simulink model "VSDk_PMSM_6"  (R2024a)
settings: Solver=VariableStepAuto  StartTime=0.0  StopTime=10.0  RelTol=1e-3
values from neighbouring files (symbols this model uses):
  faif = 0.1351    [init.m]
  Iq_limit = Tn/(1.5*p*faif)*1    (= 90.6192943499)    [init.m]
  Jm = 0.36    [init.m]
  Ki_id_vsd = Rs * wc    (= 61.7197292724)    [init.m]
  Ki_iq_vsd = Rs * wc    (= 61.7197292724)    [init.m]
  Ki_x = Rs * wc_xy    (= 61.7197292724)    [init.m]
  Ki_y = Rs * wc_xy    (= 61.7197292724)    [init.m]
  Kis_vsd = (ws^2 * Jm) / KT    (= 438.324399752)    [init.m]
  Kp_id_vsd = Ld_eff * wc    (= 0.485061905714)    [init.m]
  Kp_iq_vsd = Lq_eff * wc    (= 0.485061905714)    [init.m]
  Kp_x = Lx * wc_xy    (= 0.020106192983)    [init.m]
  Kp_y = Ly * wc_xy    (= 0.020106192983)    [init.m]
  Kps_vsd = (2 * zeta * ws * Jm) / KT    (= 19.7285507573)    [init.m]
  LD = Ld+Ldd    (= 7.72e-05)    [init.m]
  Ld = 40.2e-6    (= 4.02e-05)    [init.m]
  Ldd = 37e-6    (= 3.7e-05)    [init.m]
  Ldz = Ld-Ldd    (= 3.2e-06)    [init.m]
  LQ = Lq+Lqq    (= 7.72e-05)    [init.m]
  Lq = 40.2e-6    (= 4.02e-05)    [init.m]
  Lqq = 37e-6    (= 3.7e-05)    [init.m]
  n = 2000    [init.m]
  p = 4    [init.m]
  Rs = 9.823e-3    (= 0.009823)    [init.m]
  Tn = 734.56/10    (= 73.456)    [init.m]
  Ts = 1/(16e3)    (= 6.25e-05)    [init.m]
  Ts_FEA = 1e-7    (= 1e-07)    [init.m]
  VDC = 1200    [init.m]
  wc_xy = 2 * pi * fc_xy    (= 6283.18530718)    [init.m]
libraries: spsIGBTDiodeLib x24, spsVoltageMeasurementLib x16, spsSeriesRLCBranchLib x12, spsDiodeLib x12, spsOnDelayLib x12, slpidlib x11, simulink x7, spsControlledCurrentSourceLib x6, spsDCVoltageSourceLib x1, spsdq0toAlphaBetaZeroLib x1, spspowerguiLib x1
(part 2 of 3)

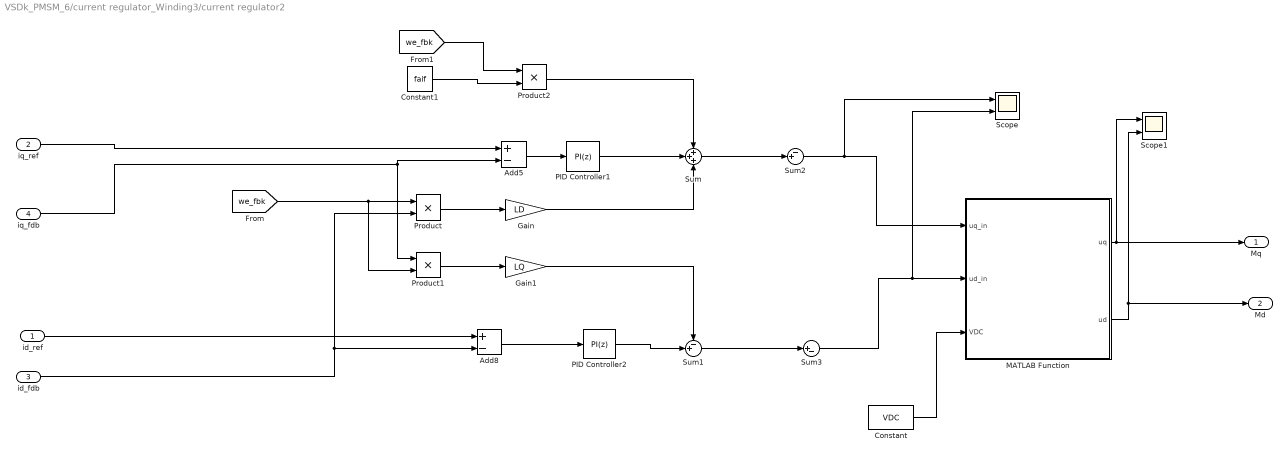
== system VSDk_PMSM_6/current regulator_Winding3/current regulator2 ==
  id_ref : Inport
  iq_ref : Inport  Port=2
  id_fdb : Inport  Port=3
  iq_fdb : Inport  Port=4
  Add5 : Sum  Inputs=+-
  Add8 : Sum  Inputs=+-
  Constant : Constant  Value=VDC
  Constant1 : Constant  Value=faif
  Gain : Gain  Gain=LD
  Gain1 : Gain  Gain=LQ
  MATLAB Function : MATLAB Function  TreatAsAtomicUnit=on
  PID Controller1 : slpidlib/PID Controller  Controller=PI  Form=Parallel  TimeDomain=Discrete-time  UseExternalTs=off  SampleTime=Ts  IntegratorMethod=Forward Euler  FilterMethod=Forward Euler  ControllerParametersSource=internal  P=Kp_iq_vsd  I=Ki_iq_vsd  UseKiTs=off  D=0  UseExternalDerivativeSource=off  N=100  UseFilter=on  TunerSelectOption=Transfer Function Based (PID Tuner App)  InitialConditionSource=internal  InitialConditionForIntegrator=0  InitialConditionForFilter=0  DifferentiatorICPrevScaledInput=0  ExternalReset=none  TrackingMode=off  Kt=1  LimitOutput=off  SatLimitsSource=internal  UpperSaturationLimit=inf  LowerSaturationLimit=-inf  LinearizeAsGain=on  AntiWindupMode=none  Kb=1  LimitIntegrator=off  UpperIntegratorSaturationLimit=inf  LowerIntegratorSaturationLimit=-inf  POutMin=[]  POutMax=[]  IOutMin=[]  IOutMax=[]  DOutMin=[]  DOutMax=[]  NOutMin=[]  NOutMax=[]  SumOutMin=[]  SumOutMax=[]  SaturationOutMin=[]  SaturationOutMax=[]  PParamMin=[]  PParamMax=[]  IParamMin=[]  IParamMax=[]  DParamMin=[]  DParamMax=[]  NParamMin=[]  NParamMax=[]  KbParamMin=[]  KbParamMax=[]  KtParamMin=[]  KtParamMax=[]  KbOutMin=[]  KbOutMax=[]  KtOutMin=[]  KtOutMax=[]  IntegratorOutMin=[]  IntegratorOutMax=[]  FilterOutMin=[]  FilterOutMax=[]  SumI1OutMin=[]  SumI1OutMax=[]  SumI2OutMin=[]  SumI2OutMax=[]  SumI3OutMin=[]  SumI3OutMax=[]  SumI4OutMin=[]  SumI4OutMax=[]  SumDOutMin=[]  SumDOutMax=[]  DifferentiatorOutMin=[]  DifferentiatorOutMax=[]  FilterDiffOutCoefMin=[]  FilterDiffOutCoefMax=[]  ReciprocalOutMin=[]  ReciprocalOutMax=[]  SumDenOutMin=[]  SumDenOutMax=[]  SumNumOutMin=[]  SumNumOutMax=[]  DivideOutMin=[]  DivideOutMax=[]  UdiffTsProdOutMin=[]  UdiffTsProdOutMax=[]  NTsProdOutMin=[]  NTsProdOutMax=[]  UintegralTsProdOutMin=[]  UintegralTsProdOutMax=[]  UngainTsProdOutMin=[]  UngainTsProdOutMax=[]  ClampingZeroOutDataTypeStr=Inherit: Inherit via back propagation  ClampingZeroOutMin=[]  ClampingZeroOutMax=[]  FilterDenConstantOutDataTypeStr=Inherit: Inherit via back propagation  FilterDenConstantOutMin=[]  FilterDenConstantOutMax=[]  PCopyOutDataTypeStr=Inherit: Inherit via back propagation  PCopyOutMin=[]  PCopyOutMax=[]  NCopyOutDataTypeStr=Inherit: Inherit via back propagation  NCopyOutMin=[]  NCopyOutMax=[]  IntegratorContinuousStateAttributes=''  IntegratorStateMustResolveToSignalObject=off  IntegratorRTWStateStorageClass=Auto  FilterContinuousStateAttributes=''  FilterStateMustResolveToSignalObject=off  FilterRTWStateStorageClass=Auto  ParallelPVariant=InternalParameters  IdealPVariant=Disabled  IVariant=InternalParameters  DVariant=Disabled  IntegratorVariant=Discrete  SatVariant=Disabled  AWVariant=Passthrough  PCopyVariant=Disabled  TRVariant=Disabled  FdbkBlocksVariant=Forward  IdealPFdbkVariant=Disabled  SatFdbkVariant=Disabled  DerivativeFilterVariant=Disabled  NVariant=Disabled  NCopyVariant=Disabled_SignalSpec  FilterICVariant=Disabled  IntegratorICVariant=InternalICs  ExternalResetVariant=Disabled  TRSumVariant=Passthrough  SumFdbkVariant=Disabled  SumVariant=Sum_PI  TsampFilterVariant=InternalTs  TsampNgainVariant=Passthrough  TsampIntegralVariant=Disabled_SignalSpec  ExternalSaturationOutDataTypeStr=Inherit: Same as second input  DerivativeSourceVariant=Disabled
  PID Controller2 : slpidlib/PID Controller  Controller=PI  Form=Parallel  TimeDomain=Discrete-time  UseExternalTs=off  SampleTime=Ts  IntegratorMethod=Forward Euler  FilterMethod=Forward Euler  ControllerParametersSource=internal  P=Kp_id_vsd  I=Ki_id_vsd  UseKiTs=off  D=0  UseExternalDerivativeSource=off  N=100  UseFilter=on  TunerSelectOption=Transfer Function Based (PID Tuner App)  InitialConditionSource=internal  InitialConditionForIntegrator=0  InitialConditionForFilter=0  DifferentiatorICPrevScaledInput=0  ExternalReset=none  TrackingMode=off  Kt=1  LimitOutput=off  SatLimitsSource=internal  UpperSaturationLimit=inf  LowerSaturationLimit=-inf  LinearizeAsGain=on  AntiWindupMode=none  Kb=1  LimitIntegrator=off  UpperIntegratorSaturationLimit=inf  LowerIntegratorSaturationLimit=-inf  POutMin=[]  POutMax=[]  IOutMin=[]  IOutMax=[]  DOutMin=[]  DOutMax=[]  NOutMin=[]  NOutMax=[]  SumOutMin=[]  SumOutMax=[]  SaturationOutMin=[]  SaturationOutMax=[]  PParamMin=[]  PParamMax=[]  IParamMin=[]  IParamMax=[]  DParamMin=[]  DParamMax=[]  NParamMin=[]  NParamMax=[]  KbParamMin=[]  KbParamMax=[]  KtParamMin=[]  KtParamMax=[]  KbOutMin=[]  KbOutMax=[]  KtOutMin=[]  KtOutMax=[]  IntegratorOutMin=[]  IntegratorOutMax=[]  FilterOutMin=[]  FilterOutMax=[]  SumI1OutMin=[]  SumI1OutMax=[]  SumI2OutMin=[]  SumI2OutMax=[]  SumI3OutMin=[]  SumI3OutMax=[]  SumI4OutMin=[]  SumI4OutMax=[]  SumDOutMin=[]  SumDOutMax=[]  DifferentiatorOutMin=[]  DifferentiatorOutMax=[]  FilterDiffOutCoefMin=[]  FilterDiffOutCoefMax=[]  ReciprocalOutMin=[]  ReciprocalOutMax=[]  SumDenOutMin=[]  SumDenOutMax=[]  SumNumOutMin=[]  SumNumOutMax=[]  DivideOutMin=[]  DivideOutMax=[]  UdiffTsProdOutMin=[]  UdiffTsProdOutMax=[]  NTsProdOutMin=[]  NTsProdOutMax=[]  UintegralTsProdOutMin=[]  UintegralTsProdOutMax=[]  UngainTsProdOutMin=[]  UngainTsProdOutMax=[]  ClampingZeroOutDataTypeStr=Inherit: Inherit via back propagation  ClampingZeroOutMin=[]  ClampingZeroOutMax=[]  FilterDenConstantOutDataTypeStr=Inherit: Inherit via back propagation  FilterDenConstantOutMin=[]  FilterDenConstantOutMax=[]  PCopyOutDataTypeStr=Inherit: Inherit via back propagation  PCopyOutMin=[]  PCopyOutMax=[]  NCopyOutDataTypeStr=Inherit: Inherit via back propagation  NCopyOutMin=[]  NCopyOutMax=[]  IntegratorContinuousStateAttributes=''  IntegratorStateMustResolveToSignalObject=off  IntegratorRTWStateStorageClass=Auto  FilterContinuousStateAttributes=''  FilterStateMustResolveToSignalObject=off  FilterRTWStateStorageClass=Auto  ParallelPVariant=InternalParameters  IdealPVariant=Disabled  IVariant=InternalParameters  DVariant=Disabled  IntegratorVariant=Discrete  SatVariant=Disabled  AWVariant=Passthrough  PCopyVariant=Disabled  TRVariant=Disabled  FdbkBlocksVariant=Forward  IdealPFdbkVariant=Disabled  SatFdbkVariant=Disabled  DerivativeFilterVariant=Disabled  NVariant=Disabled  NCopyVariant=Disabled_SignalSpec  FilterICVariant=Disabled  IntegratorICVariant=InternalICs  ExternalResetVariant=Disabled  TRSumVariant=Passthrough  SumFdbkVariant=Disabled  SumVariant=Sum_PI  TsampFilterVariant=InternalTs  TsampNgainVariant=Passthrough  TsampIntegralVariant=Disabled_SignalSpec  ExternalSaturationOutDataTypeStr=Inherit: Same as second input  DerivativeSourceVariant=Disabled
  Product : Product
  Product1 : Product
  Product2 : Product
  Scope : Scope  NumInputPorts=2
  Scope1 : Scope  NumInputPorts=2
  Sum : Sum  Inputs=+++
  Sum1 : Sum  Inputs=-+|
  Sum2 : Sum  Inputs=-+|
  Sum3 : Sum  Inputs=|+-
  Mq : Outport
  Md : Outport  Port=2
  wires:
  Constant/1 -> MATLAB Function/3(VDC)
  PID Controller1/1 -> Sum/2
  Add5/1 -> PID Controller1/1
  Add8/1 -> PID Controller2/1
  iq_ref/1 -> Add5/1
  id_ref/1 -> Add8/1
  MATLAB Function/1(uq) -> Mq/1, Scope1/1
  [we_fbk] -> Product/1, Product1/2
  Product/1 -> Gain/1
  Gain/1 -> Sum/3
  Product1/1 -> Gain1/1
  Gain1/1 -> Sum1/1
  PID Controller2/1 -> Sum1/2
  Product2/1 -> Sum/1
  [we_fbk] -> Product2/1
  Constant1/1 -> Product2/2
  Sum2/1 -> Scope/1, MATLAB Function/1(uq_in)
  Sum3/1 -> Scope/2, MATLAB Function/2(ud_in)
  Sum1/1 -> Sum3/1
  Sum/1 -> Sum2/2
  iq_fdb/1 -> Product1/1, Add5/2
  id_fdb/1 -> Add8/2, Product/2
  MATLAB Function/2(ud) -> Md/1, Scope1/2

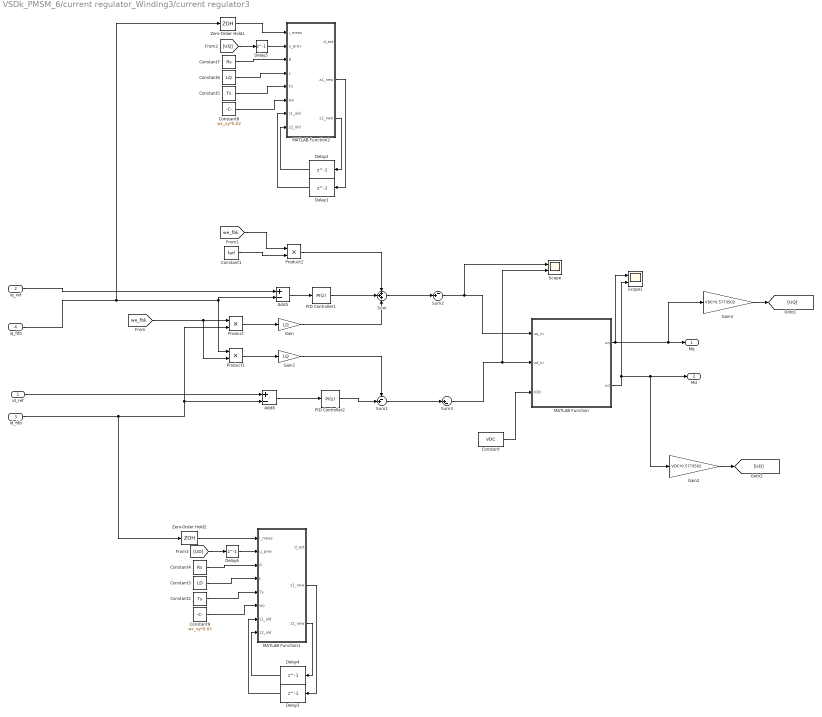
== system VSDk_PMSM_6/current regulator_Winding3/current regulator3 ==
  id_ref : Inport
  iq_ref : Inport  Port=2
  id_fdb : Inport  Port=3
  iq_fdb : Inport  Port=4
  Add5 : Sum  Inputs=+-
  Add8 : Sum  Inputs=+-
  Constant : Constant  Value=VDC
  Constant1 : Constant  Value=faif
  Constant2 : Constant  Value=Ts
  Constant3 : Constant  Value=LD
  Constant4 : Constant  Value=Rs
  Constant5 : Constant  Value=Ts
  Constant6 : Constant  Value=LQ
  Constant7 : Constant  Value=Rs
  Constant8 : Constant  Value=wc_xy*0.02
  Constant9 : Constant  Value=wc_xy*0.05
  Delay{1..6} (6 alike) : Delay  DelayLength=1  InitialCondition=0  UseCircularBuffer=on  SampleTime=Ts
  Gain : Gain  Gain=LD
  Gain1 : Gain  Gain=LQ
  Gain2 : Gain  Gain=VDC*0.5773502
  Gain3 : Gain  Gain=VDC*0.5773502
  MATLAB Function : MATLAB Function  TreatAsAtomicUnit=on
  MATLAB Function1 : MATLAB Function  TreatAsAtomicUnit=on
  MATLAB Function2 : MATLAB Function  TreatAsAtomicUnit=on
  PID Controller1 : slpidlib/PID Controller  Controller=PI  Form=Parallel  TimeDomain=Discrete-time  UseExternalTs=off  SampleTime=Ts  IntegratorMethod=Forward Euler  FilterMethod=Forward Euler  ControllerParametersSource=internal  P=Kp_iq_vsd  I=Ki_iq_vsd  UseKiTs=off  D=0  UseExternalDerivativeSource=off  N=100  UseFilter=on  TunerSelectOption=Transfer Function Based (PID Tuner App)  InitialConditionSource=internal  InitialConditionForIntegrator=0  InitialConditionForFilter=0  DifferentiatorICPrevScaledInput=0  ExternalReset=none  TrackingMode=off  Kt=1  LimitOutput=off  SatLimitsSource=internal  UpperSaturationLimit=inf  LowerSaturationLimit=-inf  LinearizeAsGain=on  AntiWindupMode=none  Kb=1  LimitIntegrator=off  UpperIntegratorSaturationLimit=inf  LowerIntegratorSaturationLimit=-inf  POutMin=[]  POutMax=[]  IOutMin=[]  IOutMax=[]  DOutMin=[]  DOutMax=[]  NOutMin=[]  NOutMax=[]  SumOutMin=[]  SumOutMax=[]  SaturationOutMin=[]  SaturationOutMax=[]  PParamMin=[]  PParamMax=[]  IParamMin=[]  IParamMax=[]  DParamMin=[]  DParamMax=[]  NParamMin=[]  NParamMax=[]  KbParamMin=[]  KbParamMax=[]  KtParamMin=[]  KtParamMax=[]  KbOutMin=[]  KbOutMax=[]  KtOutMin=[]  KtOutMax=[]  IntegratorOutMin=[]  IntegratorOutMax=[]  FilterOutMin=[]  FilterOutMax=[]  SumI1OutMin=[]  SumI1OutMax=[]  SumI2OutMin=[]  SumI2OutMax=[]  SumI3OutMin=[]  SumI3OutMax=[]  SumI4OutMin=[]  SumI4OutMax=[]  SumDOutMin=[]  SumDOutMax=[]  DifferentiatorOutMin=[]  DifferentiatorOutMax=[]  FilterDiffOutCoefMin=[]  FilterDiffOutCoefMax=[]  ReciprocalOutMin=[]  ReciprocalOutMax=[]  SumDenOutMin=[]  SumDenOutMax=[]  SumNumOutMin=[]  SumNumOutMax=[]  DivideOutMin=[]  DivideOutMax=[]  UdiffTsProdOutMin=[]  UdiffTsProdOutMax=[]  NTsProdOutMin=[]  NTsProdOutMax=[]  UintegralTsProdOutMin=[]  UintegralTsProdOutMax=[]  UngainTsProdOutMin=[]  UngainTsProdOutMax=[]  ClampingZeroOutDataTypeStr=Inherit: Inherit via back propagation  ClampingZeroOutMin=[]  ClampingZeroOutMax=[]  FilterDenConstantOutDataTypeStr=Inherit: Inherit via back propagation  FilterDenConstantOutMin=[]  FilterDenConstantOutMax=[]  PCopyOutDataTypeStr=Inherit: Inherit via back propagation  PCopyOutMin=[]  PCopyOutMax=[]  NCopyOutDataTypeStr=Inherit: Inherit via back propagation  NCopyOutMin=[]  NCopyOutMax=[]  IntegratorContinuousStateAttributes=''  IntegratorStateMustResolveToSignalObject=off  IntegratorRTWStateStorageClass=Auto  FilterContinuousStateAttributes=''  FilterStateMustResolveToSignalObject=off  FilterRTWStateStorageClass=Auto  ParallelPVariant=InternalParameters  IdealPVariant=Disabled  IVariant=InternalParameters  DVariant=Disabled  IntegratorVariant=Discrete  SatVariant=Disabled  AWVariant=Passthrough  PCopyVariant=Disabled  TRVariant=Disabled  FdbkBlocksVariant=Forward  IdealPFdbkVariant=Disabled  SatFdbkVariant=Disabled  DerivativeFilterVariant=Disabled  NVariant=Disabled  NCopyVariant=Disabled_SignalSpec  FilterICVariant=Disabled  IntegratorICVariant=InternalICs  ExternalResetVariant=Disabled  TRSumVariant=Passthrough  SumFdbkVariant=Disabled  SumVariant=Sum_PI  TsampFilterVariant=InternalTs  TsampNgainVariant=Passthrough  TsampIntegralVariant=Disabled_SignalSpec  ExternalSaturationOutDataTypeStr=Inherit: Same as second input  DerivativeSourceVariant=Disabled
  PID Controller2 : slpidlib/PID Controller  Controller=PI  Form=Parallel  TimeDomain=Discrete-time  UseExternalTs=off  SampleTime=Ts  IntegratorMethod=Forward Euler  FilterMethod=Forward Euler  ControllerParametersSource=internal  P=Kp_id_vsd  I=Ki_id_vsd  UseKiTs=off  D=0  UseExternalDerivativeSource=off  N=100  UseFilter=on  TunerSelectOption=Transfer Function Based (PID Tuner App)  InitialConditionSource=internal  InitialConditionForIntegrator=0  InitialConditionForFilter=0  DifferentiatorICPrevScaledInput=0  ExternalReset=none  TrackingMode=off  Kt=1  LimitOutput=off  SatLimitsSource=internal  UpperSaturationLimit=inf  LowerSaturationLimit=-inf  LinearizeAsGain=on  AntiWindupMode=none  Kb=1  LimitIntegrator=off  UpperIntegratorSaturationLimit=inf  LowerIntegratorSaturationLimit=-inf  POutMin=[]  POutMax=[]  IOutMin=[]  IOutMax=[]  DOutMin=[]  DOutMax=[]  NOutMin=[]  NOutMax=[]  SumOutMin=[]  SumOutMax=[]  SaturationOutMin=[]  SaturationOutMax=[]  PParamMin=[]  PParamMax=[]  IParamMin=[]  IParamMax=[]  DParamMin=[]  DParamMax=[]  NParamMin=[]  NParamMax=[]  KbParamMin=[]  KbParamMax=[]  KtParamMin=[]  KtParamMax=[]  KbOutMin=[]  KbOutMax=[]  KtOutMin=[]  KtOutMax=[]  IntegratorOutMin=[]  IntegratorOutMax=[]  FilterOutMin=[]  FilterOutMax=[]  SumI1OutMin=[]  SumI1OutMax=[]  SumI2OutMin=[]  SumI2OutMax=[]  SumI3OutMin=[]  SumI3OutMax=[]  SumI4OutMin=[]  SumI4OutMax=[]  SumDOutMin=[]  SumDOutMax=[]  DifferentiatorOutMin=[]  DifferentiatorOutMax=[]  FilterDiffOutCoefMin=[]  FilterDiffOutCoefMax=[]  ReciprocalOutMin=[]  ReciprocalOutMax=[]  SumDenOutMin=[]  SumDenOutMax=[]  SumNumOutMin=[]  SumNumOutMax=[]  DivideOutMin=[]  DivideOutMax=[]  UdiffTsProdOutMin=[]  UdiffTsProdOutMax=[]  NTsProdOutMin=[]  NTsProdOutMax=[]  UintegralTsProdOutMin=[]  UintegralTsProdOutMax=[]  UngainTsProdOutMin=[]  UngainTsProdOutMax=[]  ClampingZeroOutDataTypeStr=Inherit: Inherit via back propagation  ClampingZeroOutMin=[]  ClampingZeroOutMax=[]  FilterDenConstantOutDataTypeStr=Inherit: Inherit via back propagation  FilterDenConstantOutMin=[]  FilterDenConstantOutMax=[]  PCopyOutDataTypeStr=Inherit: Inherit via back propagation  PCopyOutMin=[]  PCopyOutMax=[]  NCopyOutDataTypeStr=Inherit: Inherit via back propagation  NCopyOutMin=[]  NCopyOutMax=[]  IntegratorContinuousStateAttributes=''  IntegratorStateMustResolveToSignalObject=off  IntegratorRTWStateStorageClass=Auto  FilterContinuousStateAttributes=''  FilterStateMustResolveToSignalObject=off  FilterRTWStateStorageClass=Auto  ParallelPVariant=InternalParameters  IdealPVariant=Disabled  IVariant=InternalParameters  DVariant=Disabled  IntegratorVariant=Discrete  SatVariant=Disabled  AWVariant=Passthrough  PCopyVariant=Disabled  TRVariant=Disabled  FdbkBlocksVariant=Forward  IdealPFdbkVariant=Disabled  SatFdbkVariant=Disabled  DerivativeFilterVariant=Disabled  NVariant=Disabled  NCopyVariant=Disabled_SignalSpec  FilterICVariant=Disabled  IntegratorICVariant=InternalICs  ExternalResetVariant=Disabled  TRSumVariant=Passthrough  SumFdbkVariant=Disabled  SumVariant=Sum_PI  TsampFilterVariant=InternalTs  TsampNgainVariant=Passthrough  TsampIntegralVariant=Disabled_SignalSpec  ExternalSaturationOutDataTypeStr=Inherit: Same as second input  DerivativeSourceVariant=Disabled
  Product : Product
  Product1 : Product
  Product2 : Product
  Scope : Scope  NumInputPorts=2
  Scope1 : Scope  NumInputPorts=2
  Sum : Sum  Inputs=+++
  Sum1 : Sum  Inputs=-+|
  Sum2 : Sum  Inputs=-+|
  Sum3 : Sum  Inputs=|+-
  Zero-Order Hold1 : ZeroOrderHold  SampleTime=Ts
  Zero-Order Hold2 : ZeroOrderHold  SampleTime=Ts
  Mq : Outport
  Md : Outport  Port=2
  wires:
  Gain3/1 -> [UQ]
  MATLAB Function/2(ud) -> Scope1/2, Md/1, Gain2/1
  Gain2/1 -> [UD]
  Delay4/1 -> MATLAB Function1/8(z2_old)
  Zero-Order Hold2/1 -> MATLAB Function1/1(i_meas)
  Constant4/1 -> MATLAB Function1/3(R)
  [UD] -> Delay6/1
  MATLAB Function1/2(z1_new) -> Delay3/1
  Delay6/1 -> MATLAB Function1/2(u_prev)
  id_fdb/1 -> Product/2, Add8/2, Zero-Order Hold2/1
  Constant2/1 -> MATLAB Function1/5(Ts)
  Delay3/1 -> MATLAB Function1/7(z1_old)
  Constant3/1 -> MATLAB Function1/4(L)
  Constant9/1 -> MATLAB Function1/6(wo)
  MATLAB Function1/3(z2_new) -> Delay4/1
  Delay2/1 -> MATLAB Function2/8(z2_old)
  Zero-Order Hold1/1 -> MATLAB Function2/1(i_meas)
  Constant7/1 -> MATLAB Function2/3(R)
  [UQ] -> Delay5/1
  MATLAB Function2/2(z1_new) -> Delay1/1
  Delay5/1 -> MATLAB Function2/2(u_prev)
  iq_fdb/1 -> Add5/2, Product1/1, Zero-Order Hold1/1
  Constant5/1 -> MATLAB Function2/5(Ts)
  Delay1/1 -> MATLAB Function2/7(z1_old)
  Constant6/1 -> MATLAB Function2/4(L)
  Constant8/1 -> MATLAB Function2/6(wo)
  MATLAB Function2/3(z2_new) -> Delay2/1
  Sum/1 -> Sum2/2
  Sum1/1 -> Sum3/1
  Sum3/1 -> MATLAB Function/2(ud_in), Scope/2
  Sum2/1 -> MATLAB Function/1(uq_in), Scope/1
  Constant1/1 -> Product2/2
  [we_fbk] -> Product2/1
  Product2/1 -> Sum/1
  PID Controller2/1 -> Sum1/2
  Gain1/1 -> Sum1/1
  Product1/1 -> Gain1/1
  Gain/1 -> Sum/3
  Product/1 -> Gain/1
  [we_fbk] -> Product1/2, Product/1
  MATLAB Function/1(uq) -> Scope1/1, Mq/1, Gain3/1
  id_ref/1 -> Add8/1
  iq_ref/1 -> Add5/1
  Add8/1 -> PID Controller2/1
  Add5/1 -> PID Controller1/1
  PID Controller1/1 -> Sum/2
  Constant/1 -> MATLAB Function/3(VDC)

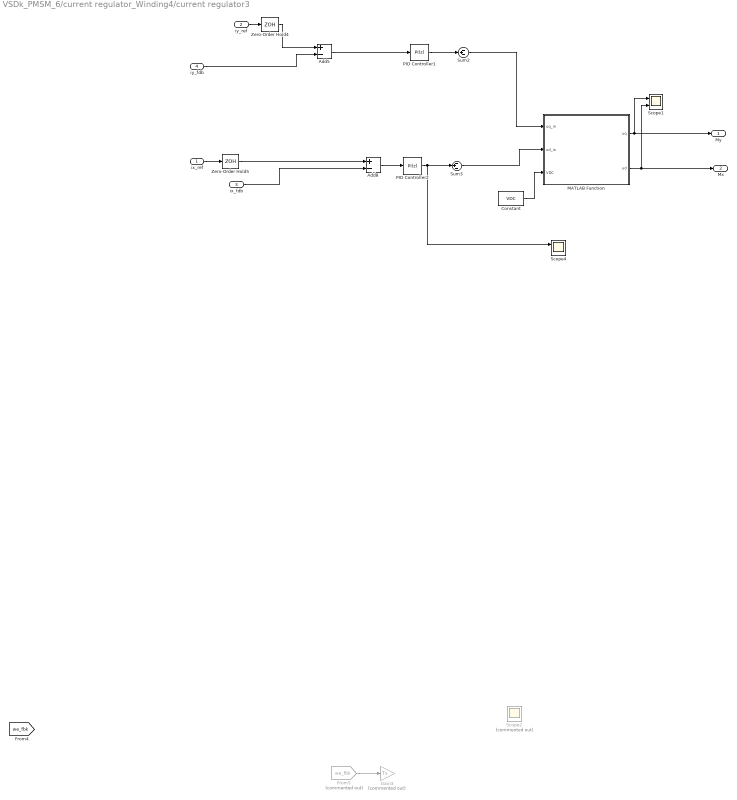
== system VSDk_PMSM_6/current regulator_Winding4/current regulator3 ==
  ix_ref : Inport
  iy_ref : Inport  Port=2
  ix_fdb : Inport  Port=3
  iy_fdb : Inport  Port=4
  Add5 : Sum  Inputs=+-
  Add8 : Sum  Inputs=+-
  Constant : Constant  Value=VDC
  From5 : From  Commented=on  GotoTag=we_fbk  TagVisibility=global
  Gain3 : Gain  Commented=on  Gain=Ts
  MATLAB Function : MATLAB Function  TreatAsAtomicUnit=on
  PID Controller1 : slpidlib/PID Controller  Controller=PI  Form=Parallel  TimeDomain=Discrete-time  UseExternalTs=off  SampleTime=Ts  IntegratorMethod=Forward Euler  FilterMethod=Forward Euler  ControllerParametersSource=internal  P=Kp_y  I=Ki_y  UseKiTs=off  D=0  UseExternalDerivativeSource=off  N=100  UseFilter=on  TunerSelectOption=Transfer Function Based (PID Tuner App)  InitialConditionSource=internal  InitialConditionForIntegrator=0  InitialConditionForFilter=0  DifferentiatorICPrevScaledInput=0  ExternalReset=none  TrackingMode=off  Kt=1  LimitOutput=off  SatLimitsSource=internal  UpperSaturationLimit=inf  LowerSaturationLimit=-inf  LinearizeAsGain=on  AntiWindupMode=none  Kb=1  LimitIntegrator=off  UpperIntegratorSaturationLimit=inf  LowerIntegratorSaturationLimit=-inf  POutMin=[]  POutMax=[]  IOutMin=[]  IOutMax=[]  DOutMin=[]  DOutMax=[]  NOutMin=[]  NOutMax=[]  SumOutMin=[]  SumOutMax=[]  SaturationOutMin=[]  SaturationOutMax=[]  PParamMin=[]  PParamMax=[]  IParamMin=[]  IParamMax=[]  DParamMin=[]  DParamMax=[]  NParamMin=[]  NParamMax=[]  KbParamMin=[]  KbParamMax=[]  KtParamMin=[]  KtParamMax=[]  KbOutMin=[]  KbOutMax=[]  KtOutMin=[]  KtOutMax=[]  IntegratorOutMin=[]  IntegratorOutMax=[]  FilterOutMin=[]  FilterOutMax=[]  SumI1OutMin=[]  SumI1OutMax=[]  SumI2OutMin=[]  SumI2OutMax=[]  SumI3OutMin=[]  SumI3OutMax=[]  SumI4OutMin=[]  SumI4OutMax=[]  SumDOutMin=[]  SumDOutMax=[]  DifferentiatorOutMin=[]  DifferentiatorOutMax=[]  FilterDiffOutCoefMin=[]  FilterDiffOutCoefMax=[]  ReciprocalOutMin=[]  ReciprocalOutMax=[]  SumDenOutMin=[]  SumDenOutMax=[]  SumNumOutMin=[]  SumNumOutMax=[]  DivideOutMin=[]  DivideOutMax=[]  UdiffTsProdOutMin=[]  UdiffTsProdOutMax=[]  NTsProdOutMin=[]  NTsProdOutMax=[]  UintegralTsProdOutMin=[]  UintegralTsProdOutMax=[]  UngainTsProdOutMin=[]  UngainTsProdOutMax=[]  ClampingZeroOutDataTypeStr=Inherit: Inherit via back propagation  ClampingZeroOutMin=[]  ClampingZeroOutMax=[]  FilterDenConstantOutDataTypeStr=Inherit: Inherit via back propagation  FilterDenConstantOutMin=[]  FilterDenConstantOutMax=[]  PCopyOutDataTypeStr=Inherit: Inherit via back propagation  PCopyOutMin=[]  PCopyOutMax=[]  NCopyOutDataTypeStr=Inherit: Inherit via back propagation  NCopyOutMin=[]  NCopyOutMax=[]  IntegratorContinuousStateAttributes=''  IntegratorStateMustResolveToSignalObject=off  IntegratorRTWStateStorageClass=Auto  FilterContinuousStateAttributes=''  FilterStateMustResolveToSignalObject=off  FilterRTWStateStorageClass=Auto  ParallelPVariant=InternalParameters  IdealPVariant=Disabled  IVariant=InternalParameters  DVariant=Disabled  IntegratorVariant=Discrete  SatVariant=Disabled  AWVariant=Passthrough  PCopyVariant=Disabled  TRVariant=Disabled  FdbkBlocksVariant=Forward  IdealPFdbkVariant=Disabled  SatFdbkVariant=Disabled  DerivativeFilterVariant=Disabled  NVariant=Disabled  NCopyVariant=Disabled_SignalSpec  FilterICVariant=Disabled  IntegratorICVariant=InternalICs  ExternalResetVariant=Disabled  TRSumVariant=Passthrough  SumFdbkVariant=Disabled  SumVariant=Sum_PI  TsampFilterVariant=InternalTs  TsampNgainVariant=Passthrough  TsampIntegralVariant=Disabled_SignalSpec  ExternalSaturationOutDataTypeStr=Inherit: Same as second input  DerivativeSourceVariant=Disabled
  PID Controller2 : slpidlib/PID Controller  Controller=PI  Form=Parallel  TimeDomain=Discrete-time  UseExternalTs=off  SampleTime=Ts  IntegratorMethod=Forward Euler  FilterMethod=Forward Euler  ControllerParametersSource=internal  P=Kp_x  I=Ki_x  UseKiTs=off  D=0  UseExternalDerivativeSource=off  N=100  UseFilter=on  TunerSelectOption=Transfer Function Based (PID Tuner App)  InitialConditionSource=internal  InitialConditionForIntegrator=0  InitialConditionForFilter=0  DifferentiatorICPrevScaledInput=0  ExternalReset=none  TrackingMode=off  Kt=1  LimitOutput=off  SatLimitsSource=internal  UpperSaturationLimit=inf  LowerSaturationLimit=-inf  LinearizeAsGain=on  AntiWindupMode=none  Kb=1  LimitIntegrator=off  UpperIntegratorSaturationLimit=inf  LowerIntegratorSaturationLimit=-inf  POutMin=[]  POutMax=[]  IOutMin=[]  IOutMax=[]  DOutMin=[]  DOutMax=[]  NOutMin=[]  NOutMax=[]  SumOutMin=[]  SumOutMax=[]  SaturationOutMin=[]  SaturationOutMax=[]  PParamMin=[]  PParamMax=[]  IParamMin=[]  IParamMax=[]  DParamMin=[]  DParamMax=[]  NParamMin=[]  NParamMax=[]  KbParamMin=[]  KbParamMax=[]  KtParamMin=[]  KtParamMax=[]  KbOutMin=[]  KbOutMax=[]  KtOutMin=[]  KtOutMax=[]  IntegratorOutMin=[]  IntegratorOutMax=[]  FilterOutMin=[]  FilterOutMax=[]  SumI1OutMin=[]  SumI1OutMax=[]  SumI2OutMin=[]  SumI2OutMax=[]  SumI3OutMin=[]  SumI3OutMax=[]  SumI4OutMin=[]  SumI4OutMax=[]  SumDOutMin=[]  SumDOutMax=[]  DifferentiatorOutMin=[]  DifferentiatorOutMax=[]  FilterDiffOutCoefMin=[]  FilterDiffOutCoefMax=[]  ReciprocalOutMin=[]  ReciprocalOutMax=[]  SumDenOutMin=[]  SumDenOutMax=[]  SumNumOutMin=[]  SumNumOutMax=[]  DivideOutMin=[]  DivideOutMax=[]  UdiffTsProdOutMin=[]  UdiffTsProdOutMax=[]  NTsProdOutMin=[]  NTsProdOutMax=[]  UintegralTsProdOutMin=[]  UintegralTsProdOutMax=[]  UngainTsProdOutMin=[]  UngainTsProdOutMax=[]  ClampingZeroOutDataTypeStr=Inherit: Inherit via back propagation  ClampingZeroOutMin=[]  ClampingZeroOutMax=[]  FilterDenConstantOutDataTypeStr=Inherit: Inherit via back propagation  FilterDenConstantOutMin=[]  FilterDenConstantOutMax=[]  PCopyOutDataTypeStr=Inherit: Inherit via back propagation  PCopyOutMin=[]  PCopyOutMax=[]  NCopyOutDataTypeStr=Inherit: Inherit via back propagation  NCopyOutMin=[]  NCopyOutMax=[]  IntegratorContinuousStateAttributes=''  IntegratorStateMustResolveToSignalObject=off  IntegratorRTWStateStorageClass=Auto  FilterContinuousStateAttributes=''  FilterStateMustResolveToSignalObject=off  FilterRTWStateStorageClass=Auto  ParallelPVariant=InternalParameters  IdealPVariant=Disabled  IVariant=InternalParameters  DVariant=Disabled  IntegratorVariant=Discrete  SatVariant=Disabled  AWVariant=Passthrough  PCopyVariant=Disabled  TRVariant=Disabled  FdbkBlocksVariant=Forward  IdealPFdbkVariant=Disabled  SatFdbkVariant=Disabled  DerivativeFilterVariant=Disabled  NVariant=Disabled  NCopyVariant=Disabled_SignalSpec  FilterICVariant=Disabled  IntegratorICVariant=InternalICs  ExternalResetVariant=Disabled  TRSumVariant=Passthrough  SumFdbkVariant=Disabled  SumVariant=Sum_PI  TsampFilterVariant=InternalTs  TsampNgainVariant=Passthrough  TsampIntegralVariant=Disabled_SignalSpec  ExternalSaturationOutDataTypeStr=Inherit: Same as second input  DerivativeSourceVariant=Disabled
  Scope1 : Scope  NumInputPorts=2
  Scope2 : Scope  Commented=on  NumInputPorts=2
  Scope4 : Scope  NumInputPorts=2
  Sum2 : Sum  Inputs=-+-
  Sum3 : Sum  Inputs=-+-
  Zero-Order Hold4 : ZeroOrderHold  SampleTime=Ts
  Zero-Order Hold5 : ZeroOrderHold  SampleTime=Ts
  My : Outport
  Mx : Outport  Port=2
  wires:
  Zero-Order Hold5/1 -> Add8/1
  Zero-Order Hold4/1 -> Add5/1
  PID Controller1/1 -> Sum2/2
  ? -> ?
  ? -> ?
  Add8/1 -> PID Controller2/1
  From5/1 -> Gain3/1
  Add5/1 -> PID Controller1/1
  MATLAB Function/2(ud) -> Scope1/2, Mx/1
  MATLAB Function/1(uq) -> Scope1/1, My/1
  PID Controller2/1 -> Sum3/2, Scope4/1
  iy_ref/1 -> Zero-Order Hold4/1
  ix_ref/1 -> Zero-Order Hold5/1
  Constant/1 -> MATLAB Function/3(VDC)
  Sum3/1 -> MATLAB Function/2(ud_in)
  Sum2/1 -> MATLAB Function/1(uq_in)
  ix_fdb/1 -> Add8/2
  iy_fdb/1 -> Add5/2

== system VSDk_PMSM_6/PMSM/Six-phae PMSM/PMSM_mechanics ==
  note: The
  note: wm
  Tm : Inport
  Te : Inport  Port=2
  1/J : Gain  Gain=1/J
  2pi : Constant  Value=2*pi
  F : Gain  Gain=F
  Integrator : Integrator
  Integrator1 : Integrator
  Mod2 : Math  Operator=mod  SignedPower=on
  Mux : Mux  Inputs=3
  Subtract : Sum  Inputs=-+-
  p : Gain  Gain=p
  m : Outport
  we : Outport  Port=2
  the : Outport  Port=3
  wires:
  Tm/1 -> Subtract/1
  Te/1 -> Subtract/2, Mux/3
  Subtract/1 -> 1/J/1
  1/J/1 -> Integrator/1
  Integrator/1 -> p/1, F/1, Mux/1
  F/1 -> Subtract/3
  p/1 -> Integrator1/1, we/1
  Integrator1/1 -> the/1, Mod2/1
  Mux/1 -> m/1
  Mod2/1 -> Mux/2
  2pi/1 -> Mod2/2

== system VSDk_PMSM_6/PMSM/Six-phae PMSM/Source ==
  uab,ubc,uuv,uvw : Inport
  we : Inport  Port=2
  the : Inport  Port=3
  Mux : Mux  Inputs=3
  Te Function : Fcn  Expr=3*p*(Flux*u[2]+(Ld-Lq)*u[1]*u[2])
  abcxyz2qdz1z2 : Subsystem
  iq,id : Subsystem
  is : Subsystem
  ix,iy : Subsystem
  m : Outport
  Te : Outport  Port=2
  wires:
  uab,ubc,uuv,uvw/1 -> abcxyz2qdz1z2/1(uab,ubc,uuv,uvw)
  the/1 -> abcxyz2qdz1z2/2(the)
  abcxyz2qdz1z2/2(ud,uq) -> iq,id/1(ud,uq)
  we/1 -> iq,id/2(we)
  abcxyz2qdz1z2/1(s,c) -> is/1(s,c)
  iq,id/1(id,iq) -> is/2(id,iq), Mux/2, Te Function/1
  Te Function/1 -> Te/1
  abcxyz2qdz1z2/3(ux,uy) -> ix,iy/1(ux,uy)
  ix,iy/1(ix,iy) -> is/3(ix,iy), Mux/3
  Mux/1 -> m/1
  is/1(is) -> Mux/1

== system VSDk_PMSM_6/PMSM/Six-phase Motor/6s//2r1 ==
  A : Inport
  B : Inport  Port=2
  C : Inport  Port=3
  U : Inport  Port=4
  V : Inport  Port=5
  W : Inport  Port=6
  theta_e : Inport  Port=7
  Fcn : Fcn  Expr=1/3*(u(1)*cos(u(7)) + u(2)*cos(u(7)-2*pi/3) + u(3)*cos(u(7)+2*pi/3) + u(4)*cos(u(7)-pi/6) + u(5)*cos(u(7)-5*pi/6) + u(6)*cos(u(7)+pi/2))
  Fcn1 : Fcn  Expr=1/3*(-u(1)*sin(u(7)) - u(2)*sin(u(7)-2*pi/3) - u(3)*sin(u(7)+2*pi/3) - u(4)*sin(u(7)-pi/6) - u(5)*sin(u(7)-5*pi/6) - u(6)*sin(u(7)+pi/2))
  Fcn2 : Fcn  Expr=1/3*(u(1) - 1/2*u(2) - 1/2*u(3) - sqrt(3)/2*u(4) + sqrt(3)/2*u(5) - 0*u(6))
  Fcn3 : Fcn  Expr=1/3*(0*u(1) - sqrt(3)/2*u(2) + sqrt(3)/2*u(3) + 1/2*u(4) + 1/2*u(5) - 1*u(6))
  Fcn4 : Fcn  Expr=1/3*(1*u(1) + 1*u(2) + 1*u(3) + 0*u(4) + 0*u(5) + 0*u(6))
  Fcn5 : Fcn  Expr=1/3*(0*u(1) + 0*u(2) + 0*u(3) + 1*u(4) + 1*u(5) + 1*u(6))
  Mux : Mux  Inputs=2
  Mux1 : Mux  Inputs=7
  Mux2 : Mux  Inputs=2
  Mux3 : Mux  Inputs=2
  Vdq : Outport
  Vxy : Outport  Port=2
  Vo1o2 : Outport  Port=3
  wires:
  Mux/1 -> Vdq/1
  Fcn1/1 -> Mux/2
  Fcn/1 -> Mux/1
  W/1 -> Mux1/6
  V/1 -> Mux1/5
  theta_e/1 -> Mux1/7
  U/1 -> Mux1/4
  C/1 -> Mux1/3
  B/1 -> Mux1/2
  A/1 -> Mux1/1
  Mux1/1 -> Fcn/1, Fcn1/1, Fcn2/1, Fcn5/1, Fcn4/1, Fcn3/1
  Mux3/1 -> Vo1o2/1
  Fcn2/1 -> Mux2/1
  Fcn3/1 -> Mux2/2
  Mux2/1 -> Vxy/1
  Fcn5/1 -> Mux3/2
  Fcn4/1 -> Mux3/1

== system VSDk_PMSM_6/PMSM/Six-phase Motor/Anti-Clark ==
  Id1 : Inport
  Iq1 : Inport  Port=2
  Id2 : Inport  Port=3
  Iq2 : Inport  Port=4
  The : Inport  Port=5
  Bus Creator{,1..3} (4 alike) : BusCreator  Inputs=3
  Fcn : Fcn  Expr=u(1)*cos(u(3))-u(2)*sin(u(3))
  Fcn1 : Fcn  Expr=u(1)*cos(u(3)-2*pi/3)-u(2)*sin(u(3)-2*pi/3)
  Fcn2 : Fcn  Expr=u(1)*cos(u(3)+2*pi/3)-u(2)*sin(u(3)+2*pi/3)
  Fcn3 : Fcn  Expr=u(2)*cos(u(1)-pi/6)-u(3)*sin(u(1)-pi/6)
  Fcn4 : Fcn  Expr=u(2)*cos(u(1)-5*pi/6)-u(3)*sin(u(1)-5*pi/6)
  Fcn5 : Fcn  Expr=u(2)*cos(u(1)+pi/2)-u(3)*sin(u(1)+pi/2)
  Iabc : Outport  VectorParamsAs1DForOutWhenUnconnected=off
  Iuvw : Outport  Port=2  VectorParamsAs1DForOutWhenUnconnected=off
  wires:
  Iq2/1 -> Bus Creator2/3
  Id2/1 -> Bus Creator2/2
  Bus Creator2/1 -> Fcn3/1, Fcn4/1, Fcn5/1
  Fcn4/1 -> Bus Creator3/2
  Fcn3/1 -> Bus Creator3/1
  Fcn5/1 -> Bus Creator3/3
  Bus Creator3/1 -> Iuvw/1
  The/1 -> Bus Creator2/1, Bus Creator/3
  Bus Creator1/1 -> Iabc/1
  Fcn2/1 -> Bus Creator1/3
  Fcn/1 -> Bus Creator1/1
  Fcn1/1 -> Bus Creator1/2
  Bus Creator/1 -> Fcn/1, Fcn1/1, Fcn2/1
  Iq1/1 -> Bus Creator/2
  Id1/1 -> Bus Creator/1

== system VSDk_PMSM_6/PMSM/Six-phase Motor/Clark ==
  Uabc : Inport
  Uvuw : Inport  Port=2
  The : Inport  Port=3
  Bus Creator{,1..3} (4 alike) : BusCreator  Inputs=2
  Fcn : Fcn  Expr=u(1)*cos(u(4))+u(2)*cos(u(4)-2*pi/3)+u(3)*cos(u(4)+2*pi/3)
  Fcn1 : Fcn  Expr=u(1)*sin(u(4))+u(2)*sin(u(4)-2*pi/3)+u(3)*sin(u(4)+2*pi/3)
  Fcn2 : Fcn  Expr=u(2)*cos(u(1)-pi/6)+u(3)*cos(u(1)-5*pi/6)+u(4)*cos(u(1)+pi/2)
  Fcn3 : Fcn  Expr=u(2)*sin(u(1)-pi/6)+u(3)*sin(u(1)-5*pi/6)+u(4)*sin(u(1)+pi/2)
  Gain : Gain  Gain=2/3
  Gain1 : Gain  Gain=-2/3
  Gain2 : Gain  Gain=2/3
  Gain3 : Gain  Gain=-2/3
  Udq1 : Outport  VectorParamsAs1DForOutWhenUnconnected=off
  Udq2 : Outport  Port=2  VectorParamsAs1DForOutWhenUnconnected=off
  wires:
  The/1 -> Bus Creator/2, Bus Creator2/1
  Bus Creator3/1 -> Udq2/1
  Gain3/1 -> Bus Creator3/2
  Gain2/1 -> Bus Creator3/1
  Uvuw/1 -> Bus Creator2/2
  Gain1/1 -> Bus Creator1/2
  Gain/1 -> Bus Creator1/1
  Bus Creator1/1 -> Udq1/1
  Uabc/1 -> Bus Creator/1
  Fcn1/1 -> Gain1/1
  Bus Creator/1 -> Fcn/1, Fcn1/1
  Fcn/1 -> Gain/1
  Bus Creator2/1 -> Fcn3/1, Fcn2/1
  Fcn2/1 -> Gain2/1
  Fcn3/1 -> Gain3/1

== system VSDk_PMSM_6/PMSM/Six-phase Motor/Machine Mode ==
  Id1 : Inport
  Iq1 : Inport  Port=2
  Id2 : Inport  Port=3
  Iq2 : Inport  Port=4
  TL : Inport  Port=5
  Bus Creator : BusCreator  Inputs=4
  Fcn : Fcn  Expr=-(Ldd-Lqq)*(u(1)+u(3))*(u(2)+u(4))+(u(2)+u(4))*Flux
  Gain : Gain  Gain=Pn*3/2
  Gain1 : Gain  Gain=Pn
  Gain2 : Gain  Gain=1/Jm
  Gain3 : Gain  Gain=B
  Integrator1 : Integrator
  Integrator2 : Integrator
  Subtract2 : Sum  Inputs=+--
  Te : Outport  VectorParamsAs1DForOutWhenUnconnected=off
  we : Outport  Port=2
  Theta : Outport  Port=3
  wires:
  Gain3/1 -> Subtract2/3
  Gain1/1 -> we/1, Integrator1/1
  Integrator2/1 -> Gain1/1, Gain3/1
  Integrator1/1 -> Theta/1
  TL/1 -> Subtract2/2
  Gain2/1 -> Integrator2/1
  Subtract2/1 -> Gain2/1
  Gain/1 -> Te/1, Subtract2/1
  Fcn/1 -> Gain/1
  Bus Creator/1 -> Fcn/1
  Iq2/1 -> Bus Creator/4
  Id1/1 -> Bus Creator/1
  Iq1/1 -> Bus Creator/2
  Id2/1 -> Bus Creator/3

== system VSDk_PMSM_6/PMSM/Six-phase Motor/Subsystem ==
  Udq1 : Inport
  Udq2 : Inport  Port=2
  We : Inport  Port=3
  Add : Sum  Inputs=+--
  Bus Creator4 : BusCreator  Inputs=2
  Demux : Demux
  Divide : Product  Inputs=/  Multiplication=Matrix(*)  RndMeth=Zero  SaturateOnIntegerOverflow=on
  Eulers Number : Constant  Value=[Rs,0,0,0;0,Rs,0,0;0,0,Rs,0;0,0,0,Rs]  OutDataTypeStr=Inherit: Inherit via back propagation
  Eulers Number1 : Constant  Value=[Ld,0,Ldd,0;0,Lq,0,Lqq;Ldd,0,Ld,0;0,Lqq,0,Lq]  OutDataTypeStr=Inherit: Inherit via back propagation
  Eulers Number2 : Constant  Value=[Flux,0,Flux,0]  VectorParams1D=off  OutDataTypeStr=Inherit: Inherit via back propagation
  Gain : Gain  Gain=[0,-1,0,0;1,0,0,0;0,0,0,-1;0,0,1,0]  Multiplication=Matrix(K*u) (u vector)
  Integrator : Integrator
  Matrix Multiply : Product  Multiplication=Matrix(*)
  Matrix Multiply1 : Product  Multiplication=Matrix(*)
  Matrix Multiply2 : Product  Multiplication=Matrix(*)
  Product : Product
  Sum : Sum  Inputs=|++
  Id1 : Outport  VectorParamsAs1DForOutWhenUnconnected=off
  Iq1 : Outport  Port=2  VectorParamsAs1DForOutWhenUnconnected=off
  Id2 : Outport  Port=3  VectorParamsAs1DForOutWhenUnconnected=off
  Iq2 : Outport  Port=4  VectorParamsAs1DForOutWhenUnconnected=off
  wires:
  Matrix Multiply1/1 -> Sum/1
  Divide/1 -> Matrix Multiply2/2
  Udq2/1 -> Bus Creator4/2
  Matrix Multiply2/1 -> Integrator/1
  Gain/1 -> Product/1
  Eulers Number1/1 -> Divide/1, Matrix Multiply1/2
  Product/1 -> Add/3
  Eulers Number2/1 -> Sum/2
  Sum/1 -> Gain/1
  Eulers Number/1 -> Matrix Multiply/2
  Add/1 -> Matrix Multiply2/1
  We/1 -> Product/2
  Matrix Multiply/1 -> Add/2
  Bus Creator4/1 -> Add/1
  Udq1/1 -> Bus Creator4/1
  Integrator/1 -> Matrix Multiply/1, Matrix Multiply1/1, Demux/1
  Demux/1 -> Id1/1
  Demux/2 -> Iq1/1
  Demux/3 -> Id2/1
  Demux/4 -> Iq2/1

== system VSDk_PMSM_6/PMSM/Six-phase Motor/is ==
  s,c : Inport
  id,iq : Inport  Port=2
  ix,iy : Inport  Port=3
  IClarke : Subsystem
  IPARK : Subsystem
  is_dq : Outport
  is_xy : Outport  Port=2
  wires:
  s,c/1 -> IPARK/1(s,c)
  id,iq/1 -> IPARK/2(id,iq)
  IPARK/1(ialpha,ibeta) -> IClarke/1(ialpha,ibeta)
  ix,iy/1 -> IClarke/2(ix,iy)
  IClarke/1(iabcuvw_dq) -> is_dq/1
  IClarke/2(iabcuvw_xy) -> is_xy/1

== system VSDk_PMSM_6/PMSM/Six-phae PMSM/Source/abcxyz2qdz1z2 ==
  uab,ubc,uuv,uvw : Inport
  the : Inport  Port=2
  Clarke : Subsystem
  Mux2 : Mux  Inputs=2
  PARK : Subsystem
  Trigonometric Function : Trigonometry
  Trigonometric Function1 : Trigonometry  Operator=cos
  s,c : Outport
  ud,uq : Outport  Port=2
  ux,uy : Outport  Port=3
  wires:
  Mux2/1 -> PARK/2(s,c), s,c/1
  the/1 -> Trigonometric Function1/1, Trigonometric Function/1
  PARK/1(ud,uq) -> ud,uq/1
  uab,ubc,uuv,uvw/1 -> Clarke/1(uab,ubc,uuv,uvw)
  Trigonometric Function1/1 -> Mux2/2
  Trigonometric Function/1 -> Mux2/1
  Clarke/1(ualpha,ubeta) -> PARK/1(ualpha,ubeta)
  Clarke/2(ux,uy) -> ux,uy/1

== system VSDk_PMSM_6/PMSM/Six-phae PMSM/Source/iq,id ==
  ud,uq : Inport
  we : Inport  Port=2
  Demux : Demux  Outputs=2
  Mux : Mux  Inputs=2
  id : Subsystem
  iq : Subsystem
  id,iq : Outport
  wires:
  ud,uq/1 -> Demux/1
  Mux/1 -> id,iq/1
  Demux/1 -> id/1(ud)
  Demux/2 -> iq/3(uq)
  we/1 -> iq/2(we), id/2(we)
  iq/1(iq) -> id/3(iq), Mux/2
  id/1(id) -> iq/1(id), Mux/1

== system VSDk_PMSM_6/PMSM/Six-phae PMSM/Source/is ==
  s,c : Inport
  id,iq : Inport  Port=2
  ix,iy : Inport  Port=3
  IClarke : Subsystem
  IPARK : Subsystem
  is : Outport
  wires:
  s,c/1 -> IPARK/1(s,c)
  id,iq/1 -> IPARK/2(id,iq)
  IPARK/1(ialpha,ibeta) -> IClarke/1(ialpha,ibeta)
  ix,iy/1 -> IClarke/2(ix,iy)
  IClarke/1(iabcuvw) -> is/1

== system VSDk_PMSM_6/PMSM/Six-phae PMSM/Source/ix,iy ==
  ux,uy : Inport
  Demux : Demux  Outputs=2
  Mux : Mux  Inputs=2
  ix : Subsystem
  iy : Subsystem
  ix,iy : Outport
  wires:
  Mux/1 -> ix,iy/1
  ux,uy/1 -> Demux/1
  Demux/1 -> ix/1(ux)
  Demux/2 -> iy/1(uy)
  ix/1(ix) -> Mux/1
  iy/1(iy) -> Mux/2

== system VSDk_PMSM_6/PMSM/Six-phase Motor/is/IClarke ==
  ialpha,ibeta : Inport
  ix,iy : Inport  Port=2
  Fcn1 : Fcn  Expr=u[1]
  Fcn10 : Fcn  Expr=-u[2]
  Fcn11 : Fcn  Expr=-1/2*u[1]+sqrt(3)/2*u[2]
  Fcn12 : Fcn  Expr=-sqrt(3)/2*u[1]+1/2*u[2]
  Fcn2 : Fcn  Expr=-1/2*u[1]+sqrt(3)/2*u[2]
  Fcn3 : Fcn  Expr=-sqrt(3)/2*u[1]+1/2*u[2]
  Fcn4 : Fcn  Expr=-u[2]
  Fcn5 : Fcn  Expr=u[1]
  Fcn6 : Fcn  Expr=-1/2*u[1]-sqrt(3)/2*u[2]
  Fcn7 : Fcn  Expr=sqrt(3)/2*u[1]+1/2*u[2]
  Fcn8 : Fcn  Expr=-1/2*u[1]-sqrt(3)/2*u[2]
  Fcn9 : Fcn  Expr=+sqrt(3)/2*u[1]+1/2*u[2]
  Mux : Mux  Inputs=6
  Mux1 : Mux  Inputs=6
  iabcuvw_dq : Outport
  iabcuvw_xy : Outport  Port=2
  wires:
  ialpha,ibeta/1 -> Fcn1/1, Fcn2/1, Fcn6/1, Fcn7/1, Fcn4/1, Fcn3/1
  Fcn1/1 -> Mux/1
  Fcn2/1 -> Mux/2
  Fcn6/1 -> Mux/3
  Fcn7/1 -> Mux/4
  Fcn3/1 -> Mux/5
  Fcn4/1 -> Mux/6
  Mux/1 -> iabcuvw_dq/1
  ix,iy/1 -> Fcn10/1, Fcn9/1, Fcn12/1, Fcn11/1, Fcn8/1, Fcn5/1
  Fcn8/1 -> Mux1/2
  Fcn12/1 -> Mux1/4
  Mux1/1 -> iabcuvw_xy/1
  Fcn9/1 -> Mux1/5
  Fcn11/1 -> Mux1/3
  Fcn10/1 -> Mux1/6
  Fcn5/1 -> Mux1/1

== system VSDk_PMSM_6/PMSM/Six-phase Motor/is/IPARK ==
  s,c : Inport
  id,iq : Inport  Port=2
  Demux : Demux  Outputs=2
  Demux1 : Demux  Outputs=2
  Mux : Mux
  Mux1 : Mux  Inputs=2
  ialpha : Fcn  Expr=u[1]*u[4]-u[2]*u[3]
  ibeta : Fcn  Expr=u[1]*u[3]+u[2]*u[4]
  ialpha,ibeta : Outport
  wires:
  Mux/1 -> ibeta/1, ialpha/1
  Demux/2 -> Mux/2
  Demux/1 -> Mux/1
  id,iq/1 -> Demux/1
  Demux1/1 -> Mux/3
  Demux1/2 -> Mux/4
  s,c/1 -> Demux1/1
  ialpha/1 -> Mux1/1
  ibeta/1 -> Mux1/2
  Mux1/1 -> ialpha,ibeta/1

== system VSDk_PMSM_6/PMSM/Six-phae PMSM/Source/abcxyz2qdz1z2/Clarke ==
  uab,ubc,uuv,uvw : Inport
  Demux : Demux
  Fcn1 : Fcn  Expr=(2*u[1]+u[2]+sqrt(3)*u[3])/6
  Fcn2 : Fcn  Expr=(sqrt(3)*u[2]+u[3]+2*u[4])/6
  Fcn6 : Fcn  Expr=(2*u[1]+u[2]-sqrt(3)*u[3])/6
  Fcn7 : Fcn  Expr=(-sqrt(3)*u[2]+u[3]+2*u[4])/6
  Mux1 : Mux  Inputs=2
  Mux2 : Mux
  Mux3 : Mux  Inputs=2
  ualpha,ubeta : Outport
  ux,uy : Outport  Port=2
  wires:
  Demux/2 -> Mux2/2
  Demux/3 -> Mux2/3
  Demux/4 -> Mux2/4
  Mux2/1 -> Fcn1/1, Fcn2/1, Fcn6/1, Fcn7/1
  uab,ubc,uuv,uvw/1 -> Demux/1
  Demux/1 -> Mux2/1
  Mux1/1 -> ualpha,ubeta/1
  Fcn1/1 -> Mux1/1
  Fcn2/1 -> Mux1/2
  Fcn6/1 -> Mux3/1
  Fcn7/1 -> Mux3/2
  Mux3/1 -> ux,uy/1

== system VSDk_PMSM_6/PMSM/Six-phae PMSM/Source/abcxyz2qdz1z2/PARK ==
  ualpha,ubeta : Inport
  s,c : Inport  Port=2
  Demux : Demux  Outputs=2
  Demux1 : Demux  Outputs=2
  Fcn : Fcn  Expr=u[1]*u[4]+u[2]*u[3]
  Fcn1 : Fcn  Expr=-u[1]*u[3]+u[2]*u[4]
  Mux : Mux
  Mux1 : Mux  Inputs=2
  ud,uq : Outport
  wires:
  Mux/1 -> Fcn/1, Fcn1/1
  s,c/1 -> Demux/1
  ualpha,ubeta/1 -> Demux1/1
  Demux1/1 -> Mux/1
  Demux1/2 -> Mux/2
  Demux/1 -> Mux/3
  Demux/2 -> Mux/4
  Fcn/1 -> Mux1/1
  Fcn1/1 -> Mux1/2
  Mux1/1 -> ud,uq/1

== system VSDk_PMSM_6/PMSM/Six-phae PMSM/Source/iq,id/id ==
  ud : Inport
  we : Inport  Port=2
  iq : Inport  Port=3
  1/Ld : Gain  Gain=1/Ld
  Lq/Ld : Gain  Gain=Lq/Ld
  Product : Product  RndMeth=Zero
  R/Ld : Gain  Gain=R/Ld
  Subtract : Sum  Inputs=-++
  d/dt(id) : Integrator
  id : Outport
  wires:
  d/dt(id)/1 -> id/1, R/Ld/1
  Subtract/1 -> d/dt(id)/1
  R/Ld/1 -> Subtract/1
  1/Ld/1 -> Subtract/2
  Lq/Ld/1 -> Subtract/3
  Product/1 -> Lq/Ld/1
  iq/1 -> Product/2
  we/1 -> Product/1
  ud/1 -> 1/Ld/1

== system VSDk_PMSM_6/PMSM/Six-phae PMSM/Source/iq,id/iq ==
  id : Inport
  we : Inport  Port=2
  uq : Inport  Port=3
  1/Lq : Gain  Gain=1/Lq
  Ld/Lq : Gain  Gain=Ld/Lq
  Product : Product  RndMeth=Zero
  R/Lq : Gain  Gain=R/Lq
  Subtract : Sum  Inputs=---+
  d/dt(iq) : Integrator
  flux/Lq : Gain  Gain=Flux/Lq
  iq : Outport
  wires:
  d/dt(iq)/1 -> iq/1, R/Lq/1
  Subtract/1 -> d/dt(iq)/1
  R/Lq/1 -> Subtract/1
  Ld/Lq/1 -> Subtract/2
  flux/Lq/1 -> Subtract/3
  1/Lq/1 -> Subtract/4
  uq/1 -> 1/Lq/1
  we/1 -> Product/2, flux/Lq/1
  id/1 -> Product/1
  Product/1 -> Ld/Lq/1

== system VSDk_PMSM_6/PMSM/Six-phae PMSM/Source/is/IClarke ==
  ialpha,ibeta : Inport
  ix,iy : Inport  Port=2
  Fcn1 : Fcn  Expr=u[1]+u[3]
  Fcn2 : Fcn  Expr=-1/2*u[1]+sqrt(3)/2*u[2]-1/2*u[3]-sqrt(3)/2*u[4]
  Fcn3 : Fcn  Expr=-sqrt(3)/2*u[1]+1/2*u[2]+sqrt(3)/2*u[3]+1/2*u[4]
  Fcn4 : Fcn  Expr=-u[2]-u[4]
  Fcn6 : Fcn  Expr=-1/2*u[1]-sqrt(3)/2*u[2]-1/2*u[3]+sqrt(3)/2*u[4]
  Fcn7 : Fcn  Expr=sqrt(3)/2*u[1]+1/2*u[2]-sqrt(3)/2*u[3]+1/2*u[4]
  Mux : Mux  Inputs=6
  Mux2 : Mux  Inputs=2
  iabcuvw : Outport
  wires:
  Mux2/1 -> Fcn1/1, Fcn2/1, Fcn6/1, Fcn7/1, Fcn4/1, Fcn3/1
  Fcn1/1 -> Mux/1
  Fcn2/1 -> Mux/2
  Fcn6/1 -> Mux/3
  Fcn7/1 -> Mux/4
  Fcn3/1 -> Mux/5
  Fcn4/1 -> Mux/6
  Mux/1 -> iabcuvw/1
  ialpha,ibeta/1 -> Mux2/1
  ix,iy/1 -> Mux2/2

== system VSDk_PMSM_6/PMSM/Six-phae PMSM/Source/is/IPARK ==
  s,c : Inport
  id,iq : Inport  Port=2
  Demux : Demux  Outputs=2
  Demux1 : Demux  Outputs=2
  Mux : Mux
  Mux1 : Mux  Inputs=2
  ialpha : Fcn  Expr=u[1]*u[4]-u[2]*u[3]
  ibeta : Fcn  Expr=u[1]*u[3]+u[2]*u[4]
  ialpha,ibeta : Outport
  wires:
  Mux/1 -> ibeta/1, ialpha/1
  Demux/2 -> Mux/2
  Demux/1 -> Mux/1
  id,iq/1 -> Demux/1
  Demux1/1 -> Mux/3
  Demux1/2 -> Mux/4
  s,c/1 -> Demux1/1
  ialpha/1 -> Mux1/1
  ibeta/1 -> Mux1/2
  Mux1/1 -> ialpha,ibeta/1

== system VSDk_PMSM_6/PMSM/Six-phae PMSM/Source/ix,iy/ix ==
  ux : Inport
  1/Lz : Gain  Gain=1/Lz
  R/Lz : Gain  Gain=R/Lz
  Subtract : Sum  Inputs=-+
  d/dt(ix) : Integrator
  ix : Outport
  tag scope: ux=global
  wires:
  d/dt(ix)/1 -> ix/1, R/Lz/1
  Subtract/1 -> d/dt(ix)/1
  R/Lz/1 -> Subtract/1
  1/Lz/1 -> Subtract/2
  ux/1 -> [ux], 1/Lz/1

== system VSDk_PMSM_6/PMSM/Six-phae PMSM/Source/ix,iy/iy ==
  uy : Inport
  1/Lz : Gain  Gain=1/Lz
  R/Lz : Gain  Gain=R/Lz
  Subtract : Sum  Inputs=-+
  d/dt(iy) : Integrator
  iy : Outport
  tag scope: uy=global
  wires:
  d/dt(iy)/1 -> iy/1, R/Lz/1
  Subtract/1 -> d/dt(iy)/1
  R/Lz/1 -> Subtract/1
  1/Lz/1 -> Subtract/2
  uy/1 -> [uy], 1/Lz/1

== matlab function VSDk_PMSM_6/Subsystem3/NTSV_9_nearest1 ==
  data: Alpha input; Beta input; Ta1 output; Ta2 output; Tb1 output; Tb2 output; Tc1 output; Tc2 output; r input; VecSector1 output
function [Ta1,Ta2,Tb1,Tb2,Tc1,Tc2,VecSector1]  = fcn(Alpha,Beta,r)
temp1=Beta;
temp2=0.8660254*Alpha+Beta*0.5;
temp3=temp2-temp1;
%0.8660254*Alpha-0.5beta
%temp1+temp2 0.8660254*Alpha+1.5beta
%temp3+temp2 2*0.8660254*Alpha
%temp1-temp3 -0.8660254*Alpha+1.5beta
VecSector1=3;
VecSector2=1;
VecSector3=0;


if temp2>0
    VecSector1=VecSector1-1;
end
if temp3>0
    VecSector1=VecSector1-1;
end
if temp1<0
    VecSector1=7-VecSector1;
end 


switch VecSector1
    case {1,4}  
       if(abs(temp2)>0.5)
           VecSector2=VecSector2+1;
           if(abs(temp3)<0.5)
               VecSector2=VecSector2+1;
               if(abs(temp1)>0.5)
                   VecSector2=VecSector2+1;
               end
           end
       end
       if(temp1<temp3)
           VecSector3=1;
       else
           VecSector3=2;
       end
    case {2,5}
       if(abs(temp1)>0.5)
           VecSector2=VecSector2+1;
           if(abs(temp2)<0.5)
               VecSector2=VecSector2+1;
               if(abs(temp3)>0.5)
                   VecSector2=VecSector2+1;
               end
           end
       end
       if(temp2+temp3>0)
          VecSector3=1;
       else
           VecSector3=2;
       end 
    case {3,6}
       if(abs(temp3)>0.5)
           VecSector2=VecSector2+1;
           if(abs(temp1)<0.5)
               VecSector2=VecSector2+1;
               if(abs(temp2)>0.5)
                   VecSector2=VecSector2+1;
               end
           end
       end
       if(temp1+temp2>0)
          VecSector3=1;
       else
           VecSector3=2;
       end 
    otherwise
        VecSector1=0;
        VecSector2=0;
end


switch VecSector1
    case 1
        Ta1=temp2;
        Ta2=1;
        Tc1=0;
        Tc2=1-temp2;
        switch VecSector2
            case 1
                Tb1=temp1;
                Tb2=1-temp3;
            case 2
                Tb1=0;
                Tb2=1+temp1-temp3;
            case 3
                Tb1=0.5-temp3;
                Tb2=0.5+temp1;
            case 4
                Tb1=temp1-temp3;
                Tb2=1;
            otherwise
                Tb1=0;
                Tb2=1;
        end
        if(VecSector3==1)
            Ta1=Ta1+Tc2*r;
            Tb2=Tb2+Tc2*r;
            Tc2=Tc2+Tc2*r;
        else
            Ta1=Ta1+Tc2*r;
            Tb1=Tb1+Tc2*r;
            Tc2=Tc2+Tc2*r;
        end
%--------------------------------------------------%
    case 2
        Tb1=temp1;
        Tb2=1;
        Tc1=0;
        Tc2=1-temp1;
        switch VecSector2
            case 1
                Ta1=temp2;
                Ta2=1+temp3;
            case 2
                Ta1=temp2+temp3;
                Ta2=1;
            case 3
                Ta1=0.5+temp3;
                Ta2=0.5+temp2;
            case 4
                Ta1=0;
                Ta2=1+temp2+temp3;
            otherwise
                Ta1=0;
                Ta2=1;
        end
        if(VecSector3==1)
            Ta1=Ta1+Tc2*r;
            Tb1=Tb1+Tc2*r;
            Tc2=Tc2+Tc2*r;
        else
            Ta2=Ta2+Tc2*r;
            Tb1=Tb1+Tc2*r;
            Tc2=Tc2+Tc2*r;
        end
%--------------------------------------------------%
    case 3
        Ta1=0;
        Ta2=1+temp3;
        Tb1=-temp3;
        Tb2=1;
        switch VecSector2
            case 1
                Tc1=-temp2;
                Tc2=1-temp1;
            case 2
                Tc1=0;
                Tc2=1-temp1-temp2;
            case 3
                Tc1=0.5-temp1;
                Tc2=0.5-temp2;
            case 4
                Tc1=-temp1-temp2;
                Tc2=1;
            otherwise
                Tc1=0;
                Tc2=1;
        end
        if(VecSector3==1)
            Tb1=Tb1+Ta2*r;
            Tc2=Tc2+Ta2*r;
            Ta2=Ta2+Ta2*r;
        else
            Tb1=Tb1+Ta2*r;
            Tc1=Tc1+Ta2*r;
            Ta2=Ta2+Ta2*r;
        end
%--------------------------------------------------%
    case 4
        Ta1=0;
        Ta2=1+temp2;
        Tc1=-temp2;
        Tc2=1;
        switch VecSector2
            case 1
                Tb1=-temp3;
                Tb2=1+temp1;
            case 2
                Tb1=temp1-temp3;
                Tb2=1;
            case 3
                Tb1=0.5+temp1;
                Tb2=0.5-temp3;
            case 4
                Tb1=0;
                Tb2=1+temp1-temp3;
            otherwise
                Tb1=0;
                Tb2=1;
        end
        if(VecSector3==1)
            Tb1=Tb1+Ta2*r;
            Tc1=Tc1+Ta2*r;
            Ta2=Ta2+Ta2*r;
        else
            Tb2=Tb2+Ta2*r;
            Tc1=Tc1+Ta2*r;
            Ta2=Ta2+Ta2*r;
        end
%--------------------------------------------------%
    case 5
        Tb1=0;
        Tb2=1+temp1;
        Tc1=-temp1;
        Tc2=1;
        switch VecSector2
            case 1
                Ta1=temp3;
                Ta2=1+temp2;
            case 2
                Ta1=0;
                Ta2=1+temp2+temp3;
            case 3
                Ta1=0.5+temp2;
                Ta2=0.5+temp3;
            case 4
                Ta1=temp2+temp3;
                Ta2=1;
            otherwise
                Ta1=0;
                Ta2=1;
        end
        if(VecSector3==1)
            Ta2=Ta2+Tb2*r;
            Tc1=Tc1+Tb2*r;
            Tb2=Tb2+Tb2*r;
        else
            Ta1=Ta1+Tb2*r;
            Tc1=Tc1+Tb2*r;
            Tb2=Tb2+Tb2*r;
        end
%--------------------------------------------------%
    case 6
        Ta1=temp3;
        Ta2=1;
        Tb1=0;
        Tb2=1-temp3;
        switch VecSector2
            case 1
                Tc1=-temp1;
                Tc2=1-temp2;
            case 2
                Tc1=-temp1-temp2;
                Tc2=1;
            case 3
                Tc1=0.5-temp2;
                Tc2=0.5-temp1;
            case 4
                Tc1=0;
                Tc2=1-temp1-temp2;
            otherwise
                Tc1=0;
                Tc2=1;
        end
        if(VecSector3==1)
            Ta1=Ta1+Tb2*r;
            Tc1=Tc1+Tb2*r;
            Tb2=Tb2+Tb2*r;
        else
            Ta1=Ta1+Tb2*r;
            Tc2=Tc2+Tb2*r;
            Tb2=Tb2+Tb2*r;
        end
%--------------------------------------------------%
    otherwise
        Ta1=0;
        Ta2=1;
        Tb1=0;
        Tb2=1;
        Tc1=0;
        Tc2=1;
end

== matlab function VSDk_PMSM_6/current regulator_Winding3/current regulator2/MATLAB Function ==
  data: uq_in input; uq output; ud_in input; ud output; VDC input
function [uq,ud] = overmodulation(uq_in,ud_in,VDC)

VDC_phase=VDC*0.5773502;
Uout=sqrt(ud_in*ud_in+uq_in*uq_in);

if(Uout>=VDC_phase*0.99)
    ud=ud_in/Uout;
    uq=uq_in/Uout;
else
    ud=ud_in/VDC_phase;
    uq=uq_in/VDC_phase;
end
end

== matlab function VSDk_PMSM_6/current regulator_Winding4/current regulator3/MATLAB Function ==
  data: uq_in input; uq output; ud_in input; ud output; VDC input
function [uq,ud] = overmodulation(uq_in,ud_in,VDC)

VDC_phase=VDC*0.5773502;
Uout=sqrt(ud_in*ud_in+uq_in*uq_in);

if(Uout>=VDC_phase*0.99)
    ud=ud_in/Uout;
    uq=uq_in/Uout;
else
    ud=ud_in/VDC_phase;
    uq=uq_in/VDC_phase;
end
end
